simulink model "gen3_pared_retira_2s"  (R2026a)
settings: Solver=ode4  StopTime=cfg.duration  FixedStep=1/(cfg.update_hz*cfg.integration_substeps)
PostLoadFcn:
  | addpath(fileparts(get_param(bdroot,'FileName'))); addpath(fileparts(fileparts(get_param(bdroot,'FileName'))));
InitFcn:
  | gen3_sl_init(bdroot);
model workspace (MAT data in the model file):
  Rd = [1  0  0; 0  1  0; 0  0  1]
  cfg.urdf = '/home/beetozp/Escritorio/MODULAR/Controlador_Impedancia/matlab/URDFFiles/GEN3_FOR_URDF_ARM_V11_MOD/urdf/GEN3_FOR_URDF_ARM_V11_MOD.urdf'
  cfg.end_effector = 'EndEffector_Link'
  cfg.q0 = [0.174532925199; 0.523598775598; -0.349065850399; 0.785398163397; 0.261799387799; -0.523598775598; 0.349065850399]
  cfg.dq0 = [0; 0; 0; 0; 0; 0; 0]
  cfg.gravity = [0 0 -9.81]
  cfg.mode = 'closed_loop'
  cfg.update_hz = 1000
  cfg.duration = 6
  cfg.integration_substeps = 4
  cfg.reference_mode = 'AbsolutePose'
  cfg.position_offset = [0.1; 0.1; -0.1]
  cfg.orientation_offset_rpy_deg = [0; 0; 0]
  cfg.absolute_position = [0.08; 0.09; -0.1]
  cfg.absolute_orientation_rpy_deg = [0; 0; 0]
  cfg.stiffness = [50; 480; 280; 10; 10; 10]
  cfg.damping_factors = [1; 1; 1; 1; 1; 1]
  cfg.enable_nullspace = 0
  cfg.nullspace_stiffness = 5
  cfg.nullspace_damping_factor = 1
  cfg.nullspace_offset = [0; 0; 0; 0; 0; 0; 0]
  cfg.enable_wrench = 0
  cfg.wrench = [0; 0; 0; 0; 0; 0]
  cfg.pose_filter = 0.1
  cfg.stiffness_filter = 1
  cfg.wrench_filter = 0.1
  cfg.nullspace_filter = 0.1
  cfg.delta_tau_max = 1
  cfg.blend_time = 2
  cfg.KTGR = [0.0889679715302; 0.0889679715302; 0.0889679715302; 0.0889679715302; 0.130890052356; 0.130890052356; 0.130890052356]
  cfg.max_current = [5; 5; 5; 5; 3; 3; 3]
  cfg.max_tau = [50.58; 50.58; 50.58; 50.58; 20.628; 20.628; 20.628]
  cfg.disturbance_tau = [0; 0; 0; 0; 0; 0; 0]
  cfg.disturbance_interval = [5 6]
  cfg.contact.enabled = 1
  cfg.contact.offset_x = 0.05
  cfg.contact.stiffness = 1500
  cfg.contact.damping = 30
  cfg.contact.active_intervals = [0 2]
  cfg.contact.reentry_ramp_s = 0
  cfg.plot = 0
  cfg.save_results = 1
  cfg.output_dir = '/home/beetozp/Escritorio/MODULAR/Controlador_Impedancia/matlab/simulink/results'
  ee = 'EndEffector_Link'
  pd = [0.08; 0.09; -0.1]
  q0 = [0.174532925199; 0.523598775598; -0.349065850399; 0.785398163397; 0.261799387799; -0.523598775598; 0.349065850399]
  robot : robotics.RigidBodyTree (value not decoded)
  wall_x = 0.672580562886
values from neighbouring files (symbols this model uses):
  cfg = gen3_release_config()    [gen3_sl_config.m]    (also in gen3_sl_init.m = gen3_sl_config(); run_gen3_simulink.m = gen3_sl_config(); validate_gen3_simulink.m = r.cfg; cfg.save_results=false; cfg.plot=false)
  robot = b.DialogPrm(1).Data    [.m]    (also in build_gen3_release_simulink.m = evalin(ws,'robot'); gen3_sl_math.m)
libraries: simulink x1
settings Model: Creator=beetozp  LastModifiedBy=beetozp

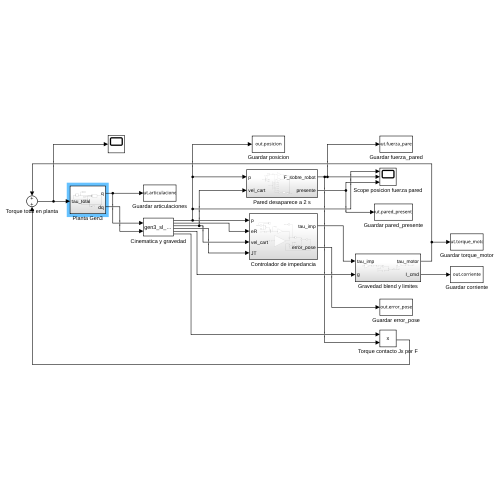
[thumbnail: Simulink's stored preview of the top-level diagram]
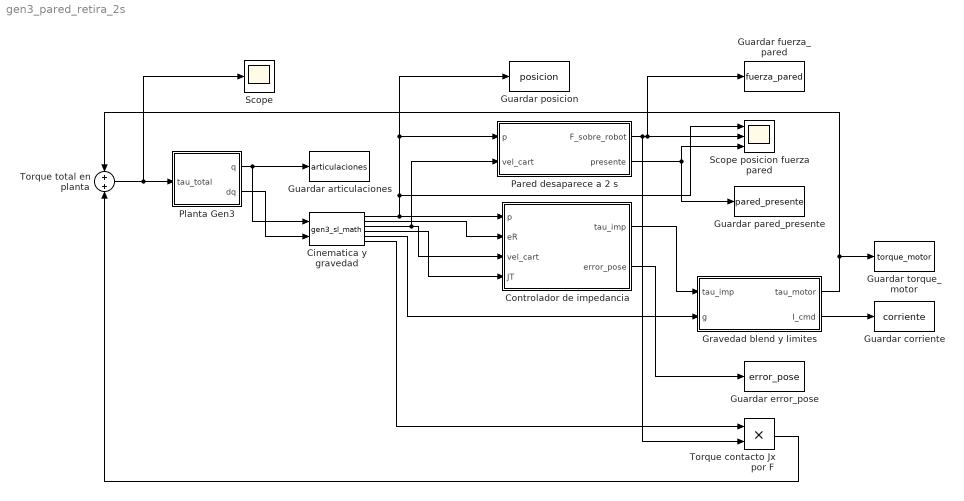
== system gen3_pared_retira_2s ==
  Cinematica y gravedad : M-S-Function  FunctionName=gen3_sl_math  Parameters=robot,Rd,'kinematics'
  Controlador de impedancia : Subsystem
  Gravedad blend y limites : Subsystem
  Guardar articulaciones : ToWorkspace  VariableName=articulaciones  SaveFormat=Timeseries  SampleTime=1/cfg.update_hz
  Guardar corriente : ToWorkspace  VariableName=corriente  SaveFormat=Timeseries  SampleTime=1/cfg.update_hz
  Guardar error_pose : ToWorkspace  VariableName=error_pose  SaveFormat=Timeseries  SampleTime=1/cfg.update_hz
  Guardar fuerza_pared : ToWorkspace  VariableName=fuerza_pared  SaveFormat=Timeseries  SampleTime=1/cfg.update_hz
  Guardar pared_presente : ToWorkspace  VariableName=pared_presente  SaveFormat=Timeseries  SampleTime=1/cfg.update_hz
  Guardar posicion : ToWorkspace  VariableName=posicion  SaveFormat=Timeseries  SampleTime=1/cfg.update_hz
  Guardar torque_motor : ToWorkspace  VariableName=torque_motor  SaveFormat=Timeseries  SampleTime=1/cfg.update_hz
  Pared desaparece a 2 s : Subsystem
  Planta Gen3 : Subsystem
  Scope : Scope
      settings: ActiveDisplayYMinimum=-63.224999999999994  ActiveDisplayYMaximum=63.224999999999994
  Scope posicion fuerza pared : Scope  NumInputPorts=3
      settings: ActiveDisplayYMinimum=-8.4518601596150553  ActiveDisplayYMaximum=2.839060138864915
  Torque contacto Jx por F : Product  Inputs=**
  Torque total en planta : Sum
  wires:
  Torque contacto Jx por F/1 -> Torque total en planta/2
  Torque total en planta/1 -> Scope/1, Planta Gen3/1(tau_total)
  Gravedad blend y limites/2(I_cmd) -> Guardar corriente/1
  Planta Gen3/1(q) -> Guardar articulaciones/1, Cinematica y gravedad/1
  Cinematica y gravedad/6 -> Torque contacto Jx por F/1
  Cinematica y gravedad/1 -> Guardar posicion/1, Pared desaparece a 2 s/1(p), Scope posicion fuerza pared/1, Controlador de impedancia/1(p)
  Cinematica y gravedad/3 -> Pared desaparece a 2 s/2(vel_cart), Controlador de impedancia/3(vel_cart)
  Cinematica y gravedad/2 -> Controlador de impedancia/2(eR)
  Gravedad blend y limites/1(tau_motor) -> Guardar torque_motor/1, Torque total en planta/1
  Cinematica y gravedad/5 -> Gravedad blend y limites/2(g)
  Planta Gen3/2(dq) -> Cinematica y gravedad/2
  Pared desaparece a 2 s/2(presente) -> Scope posicion fuerza pared/3, Guardar pared_presente/1
  Pared desaparece a 2 s/1(F_sobre_robot) -> Scope posicion fuerza pared/2, Guardar fuerza_pared/1, Torque contacto Jx por F/2
  Controlador de impedancia/1(tau_imp) -> Gravedad blend y limites/1(tau_imp)
  Cinematica y gravedad/4 -> Controlador de impedancia/4(JT)
  Controlador de impedancia/2(error_pose) -> Guardar error_pose/1

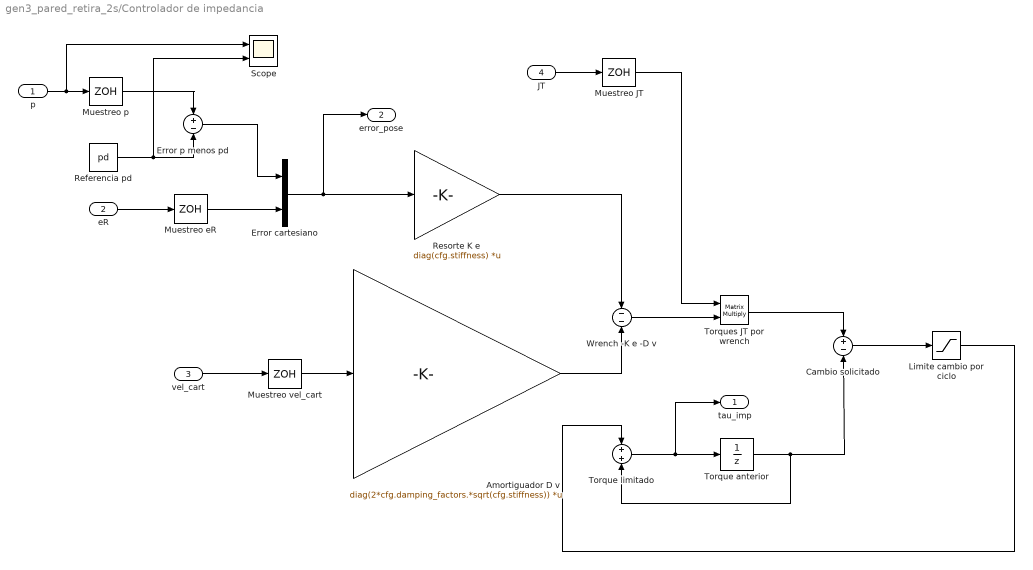
== system gen3_pared_retira_2s/Controlador de impedancia ==
  p : Inport
  eR : Inport  Port=2
  vel_cart : Inport  Port=3
  JT : Inport  Port=4
  Amortiguador D v : Gain  Gain=diag(2*cfg.damping_factors.*sqrt(cfg.stiffness))  Multiplication=Matrix(K*u)
  Cambio solicitado : Sum  Inputs=+-
  Error cartesiano : Mux  Inputs=2
  Error p menos pd : Sum  Inputs=+-
  Limite cambio por ciclo : Saturate  UpperLimit=cfg.delta_tau_max  LowerLimit=-cfg.delta_tau_max
  Muestreo JT : ZeroOrderHold  SampleTime=1/cfg.update_hz
  Muestreo eR : ZeroOrderHold  SampleTime=1/cfg.update_hz
  Muestreo p : ZeroOrderHold  SampleTime=1/cfg.update_hz
  Muestreo vel_cart : ZeroOrderHold  SampleTime=1/cfg.update_hz
  Referencia pd : Constant  Value=pd
  Resorte K e : Gain  Gain=diag(cfg.stiffness)  Multiplication=Matrix(K*u)
  Scope : Scope  NumInputPorts=2
      settings: ActiveDisplayYMinimum=-0.87497655453580969  ActiveDisplayYMaximum=1.1471791763821482  DataLoggingVariableName=ScopeData2
  Torque anterior : UnitDelay  InitialCondition=zeros(7,1)  SampleTime=1/cfg.update_hz
  Torque limitado : Sum
  Torques JT por wrench : Product  Inputs=**  Multiplication=Matrix(*)
  Wrench -K e -D v : Sum  Inputs=--
  tau_imp : Outport
  error_pose : Outport  Port=2
  wires:
  Torque anterior/1 -> Cambio solicitado/2, Torque limitado/2
  Torques JT por wrench/1 -> Cambio solicitado/1
  Torque limitado/1 -> tau_imp/1, Torque anterior/1
  Wrench -K e -D v/1 -> Torques JT por wrench/2
  Referencia pd/1 -> Scope/2, Error p menos pd/2
  Error p menos pd/1 -> Error cartesiano/1
  Muestreo JT/1 -> Torques JT por wrench/1
  eR/1 -> Muestreo eR/1
  Cambio solicitado/1 -> Limite cambio por ciclo/1
  JT/1 -> Muestreo JT/1
  Muestreo eR/1 -> Error cartesiano/2
  p/1 -> Scope/1, Muestreo p/1
  Muestreo p/1 -> Error p menos pd/1
  vel_cart/1 -> Muestreo vel_cart/1
  Error cartesiano/1 -> error_pose/1, Resorte K e/1
  Limite cambio por ciclo/1 -> Torque limitado/1
  Muestreo vel_cart/1 -> Amortiguador D v/1
  Resorte K e/1 -> Wrench -K e -D v/1
  Amortiguador D v/1 -> Wrench -K e -D v/2

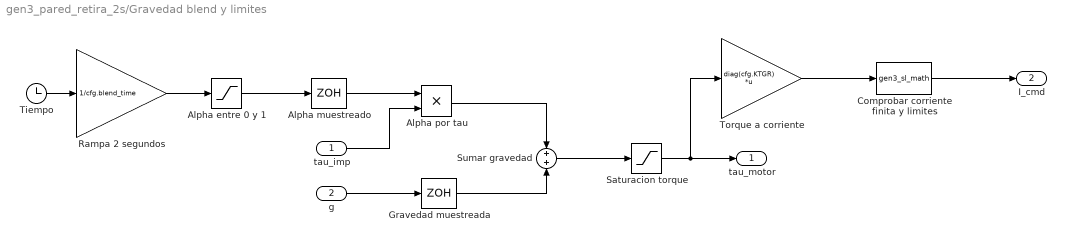
== system gen3_pared_retira_2s/Gravedad blend y limites ==
  tau_imp : Inport
  g : Inport  Port=2
  Alpha entre 0 y 1 : Saturate  UpperLimit=1  LowerLimit=0
  Alpha muestreado : ZeroOrderHold  SampleTime=1/cfg.update_hz
  Alpha por tau : Product  Inputs=**
  Comprobar corriente finita y limites : M-S-Function  FunctionName=gen3_sl_math  Parameters=cfg.max_current,cfg.KTGR,'current_check'
  Gravedad muestreada : ZeroOrderHold  SampleTime=1/cfg.update_hz
  Rampa 2 segundos : Gain  Gain=1/cfg.blend_time
  Saturacion torque : Saturate  UpperLimit=cfg.max_tau  LowerLimit=-cfg.max_tau
  Sumar gravedad : Sum
  Tiempo : Clock
  Torque a corriente : Gain  Gain=diag(cfg.KTGR)  Multiplication=Matrix(K*u)
  tau_motor : Outport
  I_cmd : Outport  Port=2
  wires:
  Saturacion torque/1 -> Torque a corriente/1, tau_motor/1
  Sumar gravedad/1 -> Saturacion torque/1
  Comprobar corriente finita y limites/1 -> I_cmd/1
  Gravedad muestreada/1 -> Sumar gravedad/2
  Alpha por tau/1 -> Sumar gravedad/1
  g/1 -> Gravedad muestreada/1
  tau_imp/1 -> Alpha por tau/2
  Alpha muestreado/1 -> Alpha por tau/1
  Alpha entre 0 y 1/1 -> Alpha muestreado/1
  Rampa 2 segundos/1 -> Alpha entre 0 y 1/1
  Torque a corriente/1 -> Comprobar corriente finita y limites/1
  Tiempo/1 -> Rampa 2 segundos/1

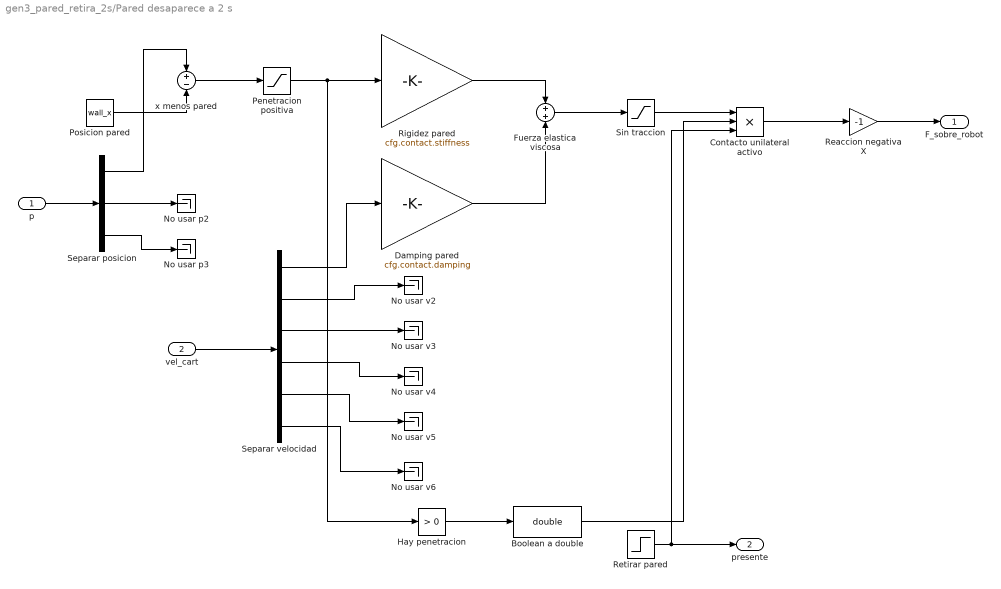
== system gen3_pared_retira_2s/Pared desaparece a 2 s ==
  p : Inport
  vel_cart : Inport  Port=2
  Boolean a double : DataTypeConversion  OutDataTypeStr=double  SaturateOnIntegerOverflow=off  RndMeth=Floor
  Contacto unilateral activo : Product  Inputs=***
  Damping pared : Gain  Gain=cfg.contact.damping
  Fuerza elastica viscosa : Sum
  Hay penetracion : simulink/Logic and Bit Operations/Compare To Constant  relop=>  const=0  OutDataTypeStr=boolean
  No usar p2 : Terminator
  No usar p3 : Terminator
  No usar v{2..6} (5 alike) : Terminator
  Penetracion positiva : Saturate  UpperLimit=inf  LowerLimit=0
  Posicion pared : Constant  Value=wall_x
  Reaccion negativa X : Gain  Gain=-1
  Retirar pared : Step  Time=2  InitialValue=1  FinalValue=0  SampleTime=0
  Rigidez pared : Gain  Gain=cfg.contact.stiffness
  Separar posicion : Demux  Outputs=3
  Separar velocidad : Demux  Outputs=6
  Sin traccion : Saturate  UpperLimit=inf  LowerLimit=0
  x menos pared : Sum  Inputs=+-
  F_sobre_robot : Outport
  presente : Outport  Port=2
  wires:
  Reaccion negativa X/1 -> F_sobre_robot/1
  Retirar pared/1 -> presente/1, Contacto unilateral activo/3
  Fuerza elastica viscosa/1 -> Sin traccion/1
  Hay penetracion/1 -> Boolean a double/1
  Damping pared/1 -> Fuerza elastica viscosa/2
  Separar velocidad/6 -> No usar v6/1
  Separar posicion/3 -> No usar p3/1
  Contacto unilateral activo/1 -> Reaccion negativa X/1
  Sin traccion/1 -> Contacto unilateral activo/1
  Penetracion positiva/1 -> Hay penetracion/1, Rigidez pared/1
  p/1 -> Separar posicion/1
  Separar posicion/1 -> x menos pared/1
  Separar posicion/2 -> No usar p2/1
  x menos pared/1 -> Penetracion positiva/1
  Rigidez pared/1 -> Fuerza elastica viscosa/1
  Separar velocidad/4 -> No usar v4/1
  vel_cart/1 -> Separar velocidad/1
  Separar velocidad/5 -> No usar v5/1
  Separar velocidad/1 -> Damping pared/1
  Posicion pared/1 -> x menos pared/2
  Separar velocidad/2 -> No usar v2/1
  Boolean a double/1 -> Contacto unilateral activo/2
  Separar velocidad/3 -> No usar v3/1

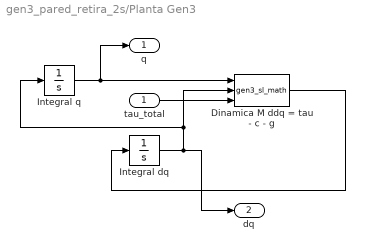
== system gen3_pared_retira_2s/Planta Gen3 ==
  tau_total : Inport
  Dinamica M ddq = tau - c - g : M-S-Function  FunctionName=gen3_sl_math  Parameters=robot,Rd,'dynamics'
  Integral dq : Integrator  InitialCondition=cfg.dq0
  Integral q : Integrator  InitialCondition=q0
  q : Outport
  dq : Outport  Port=2
  wires:
  Dinamica M ddq = tau - c - g/1 -> Integral dq/1
  Integral dq/1 -> Dinamica M ddq = tau - c - g/2, Integral q/1, dq/1
  tau_total/1 -> Dinamica M ddq = tau - c - g/3
  Integral q/1 -> q/1, Dinamica M ddq = tau - c - g/1
